simulink model "LAB_2_SMNK_przyklad"  (R2024b)
settings: Solver=ode1  StartTime=0.0  StopTime=inf  FixedStep=T  RelTol=1e-3
undefined symbols (not defined in the file): Advantech, PCI, T
libraries: sldrtlib x2, simulink x2
settings Model: SimulationMode=external  Creator=KG-MG  LastModifiedBy=Milo
settings SolverCC: AlgebraicLoopSolver=TrustRegion
settings DataIOCC: LimitDataPoints=on  SaveFormat=Array  SignalLoggingSaveFormat=ModelDataLogs  ReturnWorkspaceOutputs=off
settings OptimizationCC: ExpressionDepthLimit=2147483647  InitFltsAndDblsToZero=on
settings DebuggingCC: SaveWithParameterizedLinksMsg=none  UnderspecifiedInitializationDetection=Classic  MergeDetectMultiDrivingBlocksExec=none  SignalResolutionControl=TryResolveAllWithWarning  SolverPrmCheckMsg=warning  MultiTaskDSMMsg=warning  MultiTaskCondExecSysMsg=none  FcnCallInpInsideContextMsg=warning  UnconnectedInputMsg=warning  UnconnectedOutputMsg=warning  UnconnectedLineMsg=warning  StateNameClashWarn=warning  SFUnexpectedBacktrackingDiag=warning  SFNoUnconditionalDefaultTransitionDiag=warning  SFExecutionAtInitializationDiag=none  ArithmeticOperatorsInVariantConditions=warning
settings HardwareCC: ProdBitPerLong=64  ProdHWDeviceType=Intel->x86-64 (Linux 64)
settings ModelReferenceCC: PropagateSignalLabelsOutOfModel=off
settings SFSimCC: SimUseLocalCustomCode=off  SimParseCustomCode=off  CustomCodeUndefinedFunction=UseInterfaceOnly
settings RTWCC: Description=Simulink Desktop Real-Time  SystemTargetFile=sldrt.tlc  TemplateMakefile=sldrt.tmf  RTWUseLocalCustomCode=off  RTWCompilerOptimization=on  GPUComputeCapability=3.5
settings CodeAppCC: MaxIdLength=95  StateflowObjectComments=on
settings SimulinkDesktopRealTimeCC: TargetLibSuffix=_sldrt.a  TargetPreCompLibLocation=C:\Program Files\MATLAB\R2024b\toolbox\sldrt\lib\win64  TargetLangStandard=C89/C90 (ANSI)  ModelReferenceCompliant=off  ParMdlRefBuildCompliant=on  CompOptLevelCompliant=off  SupportVariableSizeSignals=off
settings ConfigComp: CovMetricSettings=dw  CovSaveCumulativeToWorkspaceVar=on  CovSaveSingleToWorkspaceVar=on  CovExternalEMLEnable=off

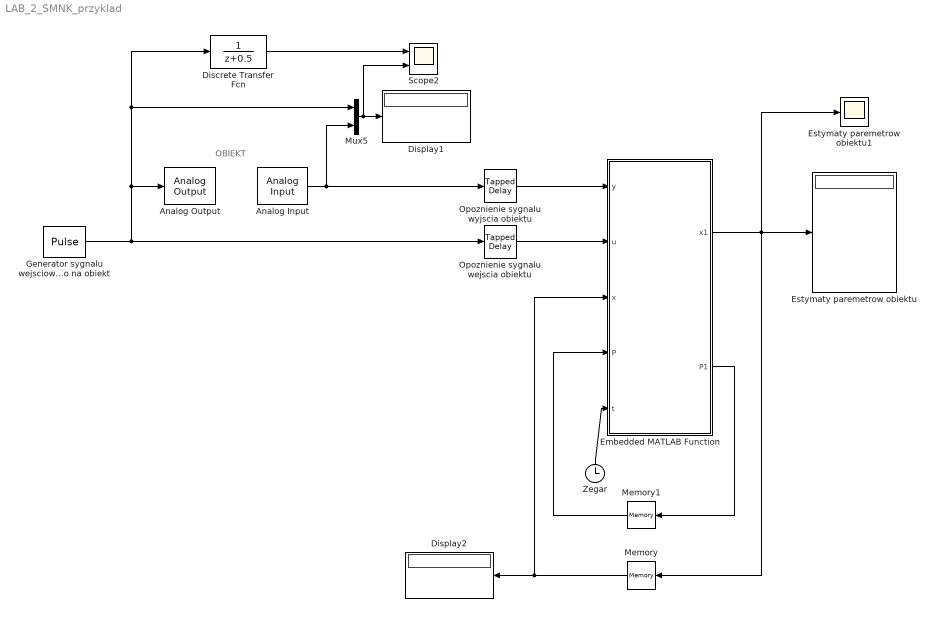
== system LAB_2_SMNK_przyklad ==
  note: OBIEKT
  " Zegar" : Clock
  Analog Input : sldrtlib/Analog Input  SampleTime=T  MaxMissedTicks=10  ShowMissedTicks=off  YieldWhenWaiting=off  DrvName=Advantech/PCI-1711  DrvAddress=4294967295  DrvOptions=zeros(1,0)  Channels=2  RangeMode=1  VoltRange=1  DataType=1
      settings: AttributesFormatString=Advantech\nPCI-1711 [auto]
  Analog Output : sldrtlib/Analog Output  SampleTime=T  MaxMissedTicks=10  ShowMissedTicks=off  YieldWhenWaiting=off  DrvName=Advantech/PCI-1711  DrvAddress=4294967295  DrvOptions=zeros(1,0)  Channels=2  RangeMode=1  VoltRange=1  InitialValue=[]  FinalValue=[]
      settings: AttributesFormatString=Advantech\nPCI-1711 [auto]
  Discrete Transfer Fcn : DiscreteTransferFcn
  Display1 : Display
  Display2 : Display
  Embedded MATLAB Function : MATLAB Function  TreatAsAtomicUnit=on
  Estymaty paremetrow obiektu : Display
  Estymaty paremetrow obiektu1 : Scope
  Generator sygnalu wejsciowego na obiekt : DiscretePulseGenerator  PulseType=Time based  Period=1  PulseWidth=50
  Memory : Memory
  Memory1 : Memory
  Mux5 : Mux  Inputs=2
  Opoznienie sygnalu wejscia obiektu : simulink/Discrete/Tapped Delay  vinit=0.0  samptime=T  NumDelays=1  DelayOrder=Oldest  includeCurrent=on
  Opoznienie sygnalu wyjscia obiektu : simulink/Discrete/Tapped Delay  vinit=0.0  samptime=T  NumDelays=1  DelayOrder=Oldest  includeCurrent=on
  Scope2 : Scope  NumInputPorts=2
  wires:
  Embedded MATLAB Function/1(x1) -> Estymaty paremetrow obiektu/1, Memory/1, Estymaty paremetrow obiektu1/1
  Memory/1 -> Display2/1, Embedded MATLAB Function/3(x)
  Opoznienie sygnalu wyjscia obiektu/1 -> Embedded MATLAB Function/1(y)
  Opoznienie sygnalu wejscia obiektu/1 -> Embedded MATLAB Function/2(u)
  " Zegar"/1 -> Embedded MATLAB Function/5(t)
  Embedded MATLAB Function/2(P1) -> Memory1/1
  Analog Input/1 -> Opoznienie sygnalu wyjscia obiektu/1, Mux5/2
  Generator sygnalu wejsciowego na obiekt/1 -> Discrete Transfer Fcn/1, Mux5/1, Analog Output/1, Opoznienie sygnalu wejscia obiektu/1
  Mux5/1 -> Display1/1, Scope2/2
  Memory1/1 -> Embedded MATLAB Function/4(P)
  Discrete Transfer Fcn/1 -> Scope2/1

== matlab function LAB_2_SMNK_przyklad/Embedded MATLAB Function ==
  settings: fimath=|
      | fimath(...
      | 'RoundMode', 'floor',...
      | 'OverflowMode', 'wrap',...
      | 'ProductMode', 'KeepLSB', 'ProductWordLength', 32,...
      | 'SumMode', 'KeepLSB', 'SumWordLength', 32,...
      | 'CastBeforeSum', false)
  data: y input; u input; x1 output; x input; P input; t input; P1 output
function [x1, P1] = fcn(y, u, x, P, t)
% WEJŚCIA:
% y - wektor [y(k-1); y(k)] z bloku Tapped Delay
% u - wektor [u(k-1); u(k)] z bloku Tapped Delay
% x - wektor estymat z poprzedniego kroku (z bloku Memory)
% P - macierz kowariancji z poprzedniego kroku (z bloku Memory1)
% t - aktualny czas symulacji (z bloku Zegar)

if t == 0 
    H = [0, 0];               % Puste H na start
    W = 1;                    % Waga
    P1 = [1000 0; 0 1000];    % Niepewność początkowa
    x1 = [0; 0];              % Parametry początkowe

else 
    % Krok k-ty > 0 (Działanie SMNK w czasie rzeczywistym)

    W = 1;

    y_stare = y(1); % y(k-1)
    y_nowe  = y(2); % y(k)
    u_nowe  = u(2); % u(k)

    % Zbudowanie wektora regresorów H = [y(k-1), u(k)]
    H = [y_stare, u_nowe];

    % Obliczenie wzmocnienia K
    Mianownik = H * P * H' + (1/W);
    K = (P * H') / Mianownik;

    % Aktualizacja macierzy kowariancji P1
    P1 = ([1 0; 0 1] - K * H) * P;

    % Aktualizacja estymat parametrów x1
    x1 = x + K * (y_nowe - H * x);
end
